simulink model "model_multicorp"  (R2026a)
settings: Solver=daessc  StopTime=0.00571428571429  MaxStep=7.93650793651e-06  RelTol=1e-9  AbsTol=1e-10
values from neighbouring files (symbols this model uses):
  C = compresor(P)    [capac.m]    (also in echilibrare.m = [0 P.r]; m02_multicorp.m = textscan(fid, ['; racire.m; s13_cinematica_fusion.m = textscan(fid, ')
  m = 3    [isg_geometrie.m]    (also in presiune_cilindru.m = u > 0 & u < 1.5)
  N = 4000    [echilibrare.m]    (also in m01_model_arbore.m = numel(th); s05_volant_activ.m = numel(th); simuleaza_arbore.m = numel(Tg))
  s = t >= t(end) - 3*60/n    [m01_model_arbore.m]    (also in racire.m = @(u) mod(-u, 360))
undefined symbols (not defined in the file or in its folder): X, Y, Z
libraries: sm_lib x21, nesl_utility x6, simulink x1
settings Model: Creator=Darian  LastModifiedBy=Darian
settings DataIOCC: OutputOption=SpecifiedOutputTimes  OutputTimes=[0 3.1746031746e-05 6.34920634921e-05 9.52380952381e-05 0.000126984126984 0.00015873015873 0.000190476190476 0.000222222222222 0.000253968253968 0.000285714285714 0.00031746031746 0.000349206349206 0.000380952380952 0.000412698412698 0.000444444444444 0.00047619047619 0.000507936507937 0.000539682539683 0.000571428571429 0.000603174603175 0.000634920634921 0.000666666666667 0.000698412698413 0.000730158730159 0.000761904761905 0.000793650793651 0.000825396825397 0.000857142857143 0.000888888888889 0.000920634920635 0.000952380952381 0.000984126984127 0.00101587301587 0.00104761904762 0.00107936507937 0.00111111111111 0.00114285714286 0.0011746031746 0.00120634920635 0.0012380952381 0.00126984126984 0.00130158730159 0.00133333333333 0.00136507936508 0.00139682539683 0.00142857142857 0.00146031746032 0.00149206349206 0.00152380952381 0.00155555555556 0.0015873015873 0.00161904761905 0.00165079365079 0.00168253968254 0.00171428571429 0.00174603174603 0.00177777777778 0.00180952380952 0.00184126984127 0.00187301587302 0.00190476190476 0.00193650793651 0.00196825396825 0.002 0.00203174603175 0.00206349206349 0.00209523809524 0.00212698412698 0.00215873015873 0.00219047619048 0.00222222222222 0.00225396825397 0.00228571428571 0.00231746031746 0.00234920634921 0.00238095238095 0.0024126984127 0.00244444444444 0.00247619047619 0.00250793650794 0.00253968253968 0.00257142857143 0.00260317460317 0.00263492063492 0.00266666666667 0.00269841269841 0.00273015873016 0.0027619047619 0.00279365079365 0.0028253968254 0.00285714285714 0.00288888888889 0.00292063492063 0.00295238095238 0.00298412698413 0.00301587301587 0.00304761904762 0.00307936507937 0.00311111111111 0.00314285714286 0.0031746031746 0.00320634920635 0.0032380952381 0.00326984126984 0.00330158730159 0.00333333333333 0.00336507936508 0.00339682539683 0.00342857142857 0.00346031746032 0.00349206349206 0.00352380952381 0.00355555555556 0.0035873015873 0.00361904761905 0.00365079365079 0.00368253968254 0.00371428571429 0.00374603174603 0.00377777777778 0.00380952380952 0.00384126984127 0.00387301587302 0.00390476190476 0.00393650793651 0.00396825396825 0.004 0.00403174603175 0.00406349206349 0.00409523809524 0.00412698412698 0.00415873015873 0.00419047619048 0.00422222222222 0.00425396825397 0.00428571428571 0.00431746031746 0.00434920634921 0.00438095238095 0.0044126984127 0.00444444444444 0.00447619047619 0.00450793650794 0.00453968253968 0.00457142857143 0.00460317460317 0.00463492063492 0.00466666666667 0.00469841269841 0.00473015873016 0.0047619047619 0.00479365079365 0.0048253968254 0.00485714285714 0.00488888888889 0.00492063492063 0.00495238095238 0.00498412698413 0.00501587301587 0.00504761904762 0.00507936507937 0.00511111111111 0.00514285714286 0.0051746031746 0.00520634920635 0.0052380952381 0.00526984126984 0.00530158730159 0.00533333333333 0.00536507936508 0.00539682539683 0.00542857142857 0.00546031746032 0.00549206349206 0.00552380952381 0.00555555555556 0.0055873015873 0.00561904761905 0.00565079365079 0.00568253968254 0.00571428571429]

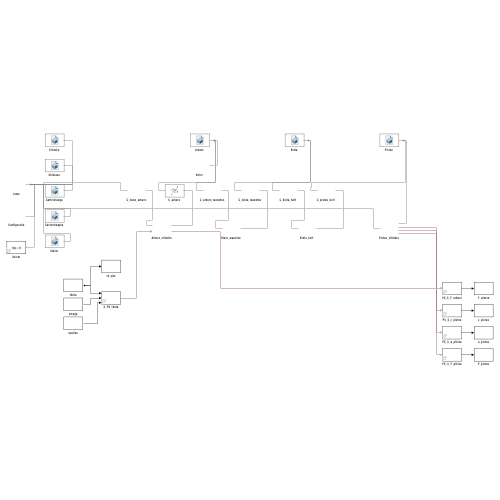
[thumbnail: Simulink's stored preview of the top-level diagram]
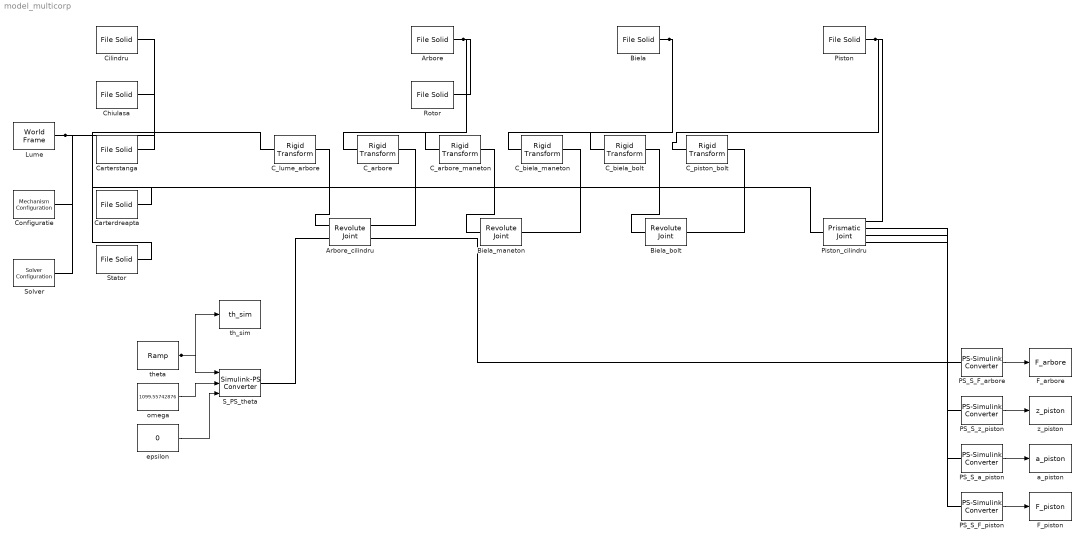
== system model_multicorp ==
  Arbore : sm_lib/Body Elements/File Solid  ExtGeomFileName=C:\Users\Darian\Documents\dizertatie_matlab\fusion\multicorp\40_Arbore.step  UnitType=FromFile  ExtGeomFileUnits=m  StepReaderType=HEX  ExportConvexHullGeometry=off  InertiaType=Custom  BasedOnType=DensityFromFile  Density=1000  DensityUnits=kg/m^3  Mass=2.277950989  MassUnits=kg  CenterOfMass=[9.035842862e-13 0.001194123027 -0.003022731061]  CenterOfMassUnits=m  MomentsOfInertia=[0.003142336917 0.001492151418 0.002716104824]  MomentsOfInertiaUnits=kg*m^2  ProductsOfInertia=[-8.580482614e-06 -8.181849604e-15 -4.711787416e-15]  ProductsOfInertiaUnits=kg*m^2  GraphicType=FromGeometry  MarkerShape=Sphere  MarkerSize=10  GraphicVisPropType=SimpleVisualProperties  GraphicDiffuseColor=[0.5 0.5 0.5]  GraphicOpacity=1  GraphicSpecularColor=[0.5 0.5 0.5 1.0]  GraphicAmbientColor=[0.15 0.15 0.15 1.0]  GraphicEmissiveColor=[0.0 0.0 0.0 1.0]  GraphicShininess=75  DoExposeReferenceFrame=on  SerializedFrames=<Frames/>
  Arbore_cilindru : sm_lib/Joints/Revolute Joint  JointMode=Normal  CompositeWrenchDir=BaseOnFollower  CompositeWrenchFrame=BaseFrame  SenseConstraintForce=off  SenseConstraintTorque=off  SenseTotalForce=on  SenseTotalTorque=off  PositionTargetSpecify=off  PositionTargetPriority=High  PositionTargetValue=0  PositionTargetValueUnits=deg  VelocityTargetSpecify=off  VelocityTargetPriority=High  VelocityTargetValue=0  VelocityTargetValueUnits=deg/s  EquilibriumPosition=0  EquilibriumPositionUnits=deg  SpringStiffness=0  SpringStiffnessUnits=N*m/deg  DampingCoefficient=0  DampingCoefficientUnits=N*m/(deg/s)  LowerLimitSpecify=off  LowerLimitBound=-90  LowerLimitBoundUnits=deg  LowerLimitStiffness=1e4  LowerLimitStiffnessUnits=N*m/deg  LowerLimitDamping=10  LowerLimitDampingUnits=N*m/(deg/s)  LowerLimitTransitionRegionWidth=0.1  LowerLimitTransitionRegionWidthUnits=deg  UpperLimitSpecify=off  UpperLimitBound=90  UpperLimitBoundUnits=deg  UpperLimitStiffness=1e4  UpperLimitStiffnessUnits=N*m/deg  UpperLimitDamping=10  UpperLimitDampingUnits=N*m/(deg/s)  UpperLimitTransitionRegionWidth=0.1  UpperLimitTransitionRegionWidthUnits=deg  TorqueActuationMode=ComputedTorque  MotionActuationMode=InputMotion  SensePosition=off  SenseVelocity=off  SenseAcceleration=off  SenseTorqueForce=off  SenseLowerLimitTorqueForce=off  SenseUpperLimitTorqueForce=off
  Biela : sm_lib/Body Elements/File Solid  ExtGeomFileName=C:\Users\Darian\Documents\dizertatie_matlab\fusion\multicorp\30_Biela.step  UnitType=FromFile  ExtGeomFileUnits=m  StepReaderType=HEX  ExportConvexHullGeometry=off  InertiaType=Custom  BasedOnType=DensityFromFile  Density=1000  DensityUnits=kg/m^3  Mass=0.181830075  MassUnits=kg  CenterOfMass=[-3.952804341e-13 -7.668919001e-19 0.0693849363]  CenterOfMassUnits=m  MomentsOfInertia=[0.0003677202797 0.0003764850798 1.5782604e-05]  MomentsOfInertiaUnits=kg*m^2  ProductsOfInertia=[-1.839056463e-20 -1.125578697e-15 -4.183320357e-21]  ProductsOfInertiaUnits=kg*m^2  GraphicType=FromGeometry  MarkerShape=Sphere  MarkerSize=10  GraphicVisPropType=SimpleVisualProperties  GraphicDiffuseColor=[0.5 0.5 0.5]  GraphicOpacity=1  GraphicSpecularColor=[0.5 0.5 0.5 1.0]  GraphicAmbientColor=[0.15 0.15 0.15 1.0]  GraphicEmissiveColor=[0.0 0.0 0.0 1.0]  GraphicShininess=75  DoExposeReferenceFrame=on  SerializedFrames=<Frames/>
  Biela_bolt : sm_lib/Joints/Revolute Joint  JointMode=Normal  CompositeWrenchDir=FollowerOnBase  CompositeWrenchFrame=BaseFrame  SenseConstraintForce=off  SenseConstraintTorque=off  SenseTotalForce=off  SenseTotalTorque=off  PositionTargetSpecify=off  PositionTargetPriority=High  PositionTargetValue=0  PositionTargetValueUnits=deg  VelocityTargetSpecify=off  VelocityTargetPriority=High  VelocityTargetValue=0  VelocityTargetValueUnits=deg/s  EquilibriumPosition=0  EquilibriumPositionUnits=deg  SpringStiffness=0  SpringStiffnessUnits=N*m/deg  DampingCoefficient=0  DampingCoefficientUnits=N*m/(deg/s)  LowerLimitSpecify=off  LowerLimitBound=-90  LowerLimitBoundUnits=deg  LowerLimitStiffness=1e4  LowerLimitStiffnessUnits=N*m/deg  LowerLimitDamping=10  LowerLimitDampingUnits=N*m/(deg/s)  LowerLimitTransitionRegionWidth=0.1  LowerLimitTransitionRegionWidthUnits=deg  UpperLimitSpecify=off  UpperLimitBound=90  UpperLimitBoundUnits=deg  UpperLimitStiffness=1e4  UpperLimitStiffnessUnits=N*m/deg  UpperLimitDamping=10  UpperLimitDampingUnits=N*m/(deg/s)  UpperLimitTransitionRegionWidth=0.1  UpperLimitTransitionRegionWidthUnits=deg  TorqueActuationMode=NoTorque  MotionActuationMode=ComputedMotion  SensePosition=off  SenseVelocity=off  SenseAcceleration=off  SenseTorqueForce=off  SenseLowerLimitTorqueForce=off  SenseUpperLimitTorqueForce=off
  Biela_maneton : sm_lib/Joints/Revolute Joint  JointMode=Normal  CompositeWrenchDir=FollowerOnBase  CompositeWrenchFrame=BaseFrame  SenseConstraintForce=off  SenseConstraintTorque=off  SenseTotalForce=off  SenseTotalTorque=off  PositionTargetSpecify=off  PositionTargetPriority=High  PositionTargetValue=0  PositionTargetValueUnits=deg  VelocityTargetSpecify=off  VelocityTargetPriority=High  VelocityTargetValue=0  VelocityTargetValueUnits=deg/s  EquilibriumPosition=0  EquilibriumPositionUnits=deg  SpringStiffness=0  SpringStiffnessUnits=N*m/deg  DampingCoefficient=0  DampingCoefficientUnits=N*m/(deg/s)  LowerLimitSpecify=off  LowerLimitBound=-90  LowerLimitBoundUnits=deg  LowerLimitStiffness=1e4  LowerLimitStiffnessUnits=N*m/deg  LowerLimitDamping=10  LowerLimitDampingUnits=N*m/(deg/s)  LowerLimitTransitionRegionWidth=0.1  LowerLimitTransitionRegionWidthUnits=deg  UpperLimitSpecify=off  UpperLimitBound=90  UpperLimitBoundUnits=deg  UpperLimitStiffness=1e4  UpperLimitStiffnessUnits=N*m/deg  UpperLimitDamping=10  UpperLimitDampingUnits=N*m/(deg/s)  UpperLimitTransitionRegionWidth=0.1  UpperLimitTransitionRegionWidthUnits=deg  TorqueActuationMode=NoTorque  MotionActuationMode=ComputedMotion  SensePosition=off  SenseVelocity=off  SenseAcceleration=off  SenseTorqueForce=off  SenseLowerLimitTorqueForce=off  SenseUpperLimitTorqueForce=off
  C_arbore : sm_lib/Frames and Transforms/Rigid Transform  RotationMethod=StandardAxis  FollAlignAxisA=+X  BaseAlignAxisA=+Y  FollAlignAxisB=+Y  BaseAlignAxisB=+Z  RotationStandardAxis=+X  RotationAngle=-90  RotationAngleUnits=deg  RotationArbitraryAxis=[0 0 1]  RotationSequenceAxes=FollowerAxes  RotationSequence=XYX  RotationSequenceAngles=[0 0 0]  RotationSequenceAnglesUnits=deg  RotationMatrix=[1 0 0;0 1 0;0 0 1]  Quaternion=[1 0 0 0]  TranslationMethod=Cartesian  TranslationCartesianOffset=[0 0 0]  TranslationCartesianOffsetUnits=m  TranslationStandardAxis=+Z  TranslationStandardOffset=0  TranslationStandardOffsetUnits=m  TranslationROffset=0  TranslationROffsetUnits=m  TranslationThetaOffset=0  TranslationThetaOffsetUnits=deg  TranslationZOffset=0  TranslationZOffsetUnits=m
  C_arbore_maneton : sm_lib/Frames and Transforms/Rigid Transform  RotationMethod=StandardAxis  FollAlignAxisA=+X  BaseAlignAxisA=+Y  FollAlignAxisB=+Y  BaseAlignAxisB=+Z  RotationStandardAxis=+X  RotationAngle=-90  RotationAngleUnits=deg  RotationArbitraryAxis=[0 0 1]  RotationSequenceAxes=FollowerAxes  RotationSequence=XYX  RotationSequenceAngles=[0 0 0]  RotationSequenceAnglesUnits=deg  RotationMatrix=[1 0 0;0 1 0;0 0 1]  Quaternion=[1 0 0 0]  TranslationMethod=Cartesian  TranslationCartesianOffset=[0 0 0.02725]  TranslationCartesianOffsetUnits=m  TranslationStandardAxis=+Z  TranslationStandardOffset=0  TranslationStandardOffsetUnits=m  TranslationROffset=0  TranslationROffsetUnits=m  TranslationThetaOffset=0  TranslationThetaOffsetUnits=deg  TranslationZOffset=0  TranslationZOffsetUnits=m
  C_biela_bolt : sm_lib/Frames and Transforms/Rigid Transform  RotationMethod=StandardAxis  FollAlignAxisA=+X  BaseAlignAxisA=+Y  FollAlignAxisB=+Y  BaseAlignAxisB=+Z  RotationStandardAxis=+X  RotationAngle=-90  RotationAngleUnits=deg  RotationArbitraryAxis=[0 0 1]  RotationSequenceAxes=FollowerAxes  RotationSequence=XYX  RotationSequenceAngles=[0 0 0]  RotationSequenceAnglesUnits=deg  RotationMatrix=[1 0 0;0 1 0;0 0 1]  Quaternion=[1 0 0 0]  TranslationMethod=Cartesian  TranslationCartesianOffset=[0 0 0.13725]  TranslationCartesianOffsetUnits=m  TranslationStandardAxis=+Z  TranslationStandardOffset=0  TranslationStandardOffsetUnits=m  TranslationROffset=0  TranslationROffsetUnits=m  TranslationThetaOffset=0  TranslationThetaOffsetUnits=deg  TranslationZOffset=0  TranslationZOffsetUnits=m
  C_biela_maneton : sm_lib/Frames and Transforms/Rigid Transform  RotationMethod=StandardAxis  FollAlignAxisA=+X  BaseAlignAxisA=+Y  FollAlignAxisB=+Y  BaseAlignAxisB=+Z  RotationStandardAxis=+X  RotationAngle=-90  RotationAngleUnits=deg  RotationArbitraryAxis=[0 0 1]  RotationSequenceAxes=FollowerAxes  RotationSequence=XYX  RotationSequenceAngles=[0 0 0]  RotationSequenceAnglesUnits=deg  RotationMatrix=[1 0 0;0 1 0;0 0 1]  Quaternion=[1 0 0 0]  TranslationMethod=Cartesian  TranslationCartesianOffset=[0 0 0.02725]  TranslationCartesianOffsetUnits=m  TranslationStandardAxis=+Z  TranslationStandardOffset=0  TranslationStandardOffsetUnits=m  TranslationROffset=0  TranslationROffsetUnits=m  TranslationThetaOffset=0  TranslationThetaOffsetUnits=deg  TranslationZOffset=0  TranslationZOffsetUnits=m
  C_lume_arbore : sm_lib/Frames and Transforms/Rigid Transform  RotationMethod=StandardAxis  FollAlignAxisA=+X  BaseAlignAxisA=+Y  FollAlignAxisB=+Y  BaseAlignAxisB=+Z  RotationStandardAxis=+X  RotationAngle=-90  RotationAngleUnits=deg  RotationArbitraryAxis=[0 0 1]  RotationSequenceAxes=FollowerAxes  RotationSequence=XYX  RotationSequenceAngles=[0 0 0]  RotationSequenceAnglesUnits=deg  RotationMatrix=[1 0 0;0 1 0;0 0 1]  Quaternion=[1 0 0 0]  TranslationMethod=Cartesian  TranslationCartesianOffset=[0 0 0]  TranslationCartesianOffsetUnits=m  TranslationStandardAxis=+Z  TranslationStandardOffset=0  TranslationStandardOffsetUnits=m  TranslationROffset=0  TranslationROffsetUnits=m  TranslationThetaOffset=0  TranslationThetaOffsetUnits=deg  TranslationZOffset=0  TranslationZOffsetUnits=m
  C_piston_bolt : sm_lib/Frames and Transforms/Rigid Transform  RotationMethod=StandardAxis  FollAlignAxisA=+X  BaseAlignAxisA=+Y  FollAlignAxisB=+Y  BaseAlignAxisB=+Z  RotationStandardAxis=+X  RotationAngle=-90  RotationAngleUnits=deg  RotationArbitraryAxis=[0 0 1]  RotationSequenceAxes=FollowerAxes  RotationSequence=XYX  RotationSequenceAngles=[0 0 0]  RotationSequenceAnglesUnits=deg  RotationMatrix=[1 0 0;0 1 0;0 0 1]  Quaternion=[1 0 0 0]  TranslationMethod=Cartesian  TranslationCartesianOffset=[0 0 0.13725]  TranslationCartesianOffsetUnits=m  TranslationStandardAxis=+Z  TranslationStandardOffset=0  TranslationStandardOffsetUnits=m  TranslationROffset=0  TranslationROffsetUnits=m  TranslationThetaOffset=0  TranslationThetaOffsetUnits=deg  TranslationZOffset=0  TranslationZOffsetUnits=m
  Carterdreapta : sm_lib/Body Elements/File Solid  ExtGeomFileName=C:\Users\Darian\Documents\dizertatie_matlab\fusion\multicorp\51_Carter_dreapta.step  UnitType=FromFile  ExtGeomFileUnits=m  StepReaderType=HEX  ExportConvexHullGeometry=off  InertiaType=Custom  BasedOnType=DensityFromFile  Density=1000  DensityUnits=kg/m^3  Mass=1  MassUnits=kg  CenterOfMass=[0 0 0]  CenterOfMassUnits=m  MomentsOfInertia=[1 1 1]*1e-3  MomentsOfInertiaUnits=kg*m^2  ProductsOfInertia=[0 0 0]  ProductsOfInertiaUnits=kg*m^2  GraphicType=FromGeometry  MarkerShape=Sphere  MarkerSize=10  GraphicVisPropType=AdvancedVisualProperties  GraphicDiffuseColor=[0.5 0.5 0.5]  GraphicOpacity=0.25  GraphicSpecularColor=[0.5 0.5 0.5 1.0]  GraphicAmbientColor=[0.15 0.15 0.15 1.0]  GraphicEmissiveColor=[0.0 0.0 0.0 1.0]  GraphicShininess=75  DoExposeReferenceFrame=on  SerializedFrames=<Frames/>
  Carterstanga : sm_lib/Body Elements/File Solid  ExtGeomFileName=C:\Users\Darian\Documents\dizertatie_matlab\fusion\multicorp\50_Carter_stanga.step  UnitType=FromFile  ExtGeomFileUnits=m  StepReaderType=HEX  ExportConvexHullGeometry=off  InertiaType=Custom  BasedOnType=DensityFromFile  Density=1000  DensityUnits=kg/m^3  Mass=1  MassUnits=kg  CenterOfMass=[0 0 0]  CenterOfMassUnits=m  MomentsOfInertia=[1 1 1]*1e-3  MomentsOfInertiaUnits=kg*m^2  ProductsOfInertia=[0 0 0]  ProductsOfInertiaUnits=kg*m^2  GraphicType=FromGeometry  MarkerShape=Sphere  MarkerSize=10  GraphicVisPropType=AdvancedVisualProperties  GraphicDiffuseColor=[0.5 0.5 0.5]  GraphicOpacity=0.25  GraphicSpecularColor=[0.5 0.5 0.5 1.0]  GraphicAmbientColor=[0.15 0.15 0.15 1.0]  GraphicEmissiveColor=[0.0 0.0 0.0 1.0]  GraphicShininess=75  DoExposeReferenceFrame=on  SerializedFrames=<Frames/>
  Chiulasa : sm_lib/Body Elements/File Solid  ExtGeomFileName=C:\Users\Darian\Documents\dizertatie_matlab\fusion\multicorp\15_Chiulasa.step  UnitType=FromFile  ExtGeomFileUnits=m  StepReaderType=HEX  ExportConvexHullGeometry=off  InertiaType=Custom  BasedOnType=DensityFromFile  Density=1000  DensityUnits=kg/m^3  Mass=1  MassUnits=kg  CenterOfMass=[0 0 0]  CenterOfMassUnits=m  MomentsOfInertia=[1 1 1]*1e-3  MomentsOfInertiaUnits=kg*m^2  ProductsOfInertia=[0 0 0]  ProductsOfInertiaUnits=kg*m^2  GraphicType=FromGeometry  MarkerShape=Sphere  MarkerSize=10  GraphicVisPropType=AdvancedVisualProperties  GraphicDiffuseColor=[0.5 0.5 0.5]  GraphicOpacity=0.25  GraphicSpecularColor=[0.5 0.5 0.5 1.0]  GraphicAmbientColor=[0.15 0.15 0.15 1.0]  GraphicEmissiveColor=[0.0 0.0 0.0 1.0]  GraphicShininess=75  DoExposeReferenceFrame=on  SerializedFrames=<Frames/>
  Cilindru : sm_lib/Body Elements/File Solid  ExtGeomFileName=C:\Users\Darian\Documents\dizertatie_matlab\fusion\multicorp\10_Cilindru.step  UnitType=FromFile  ExtGeomFileUnits=m  StepReaderType=HEX  ExportConvexHullGeometry=off  InertiaType=Custom  BasedOnType=DensityFromFile  Density=1000  DensityUnits=kg/m^3  Mass=1  MassUnits=kg  CenterOfMass=[0 0 0]  CenterOfMassUnits=m  MomentsOfInertia=[1 1 1]*1e-3  MomentsOfInertiaUnits=kg*m^2  ProductsOfInertia=[0 0 0]  ProductsOfInertiaUnits=kg*m^2  GraphicType=FromGeometry  MarkerShape=Sphere  MarkerSize=10  GraphicVisPropType=AdvancedVisualProperties  GraphicDiffuseColor=[0.5 0.5 0.5]  GraphicOpacity=0.25  GraphicSpecularColor=[0.5 0.5 0.5 1.0]  GraphicAmbientColor=[0.15 0.15 0.15 1.0]  GraphicEmissiveColor=[0.0 0.0 0.0 1.0]  GraphicShininess=75  DoExposeReferenceFrame=on  SerializedFrames=<Frames/>
  Configuratie : sm_lib/Utilities/Mechanism Configuration  UniformGravity=None  GravityVector=[0 0 -9.80665]  GravityVectorUnits=m/s^2  LinearizationDelta=0.001  JointModeTransitionNonlinearIterations=2
  F_arbore : ToWorkspace  VariableName=F_arbore  SampleTime=-1
  F_piston : ToWorkspace  VariableName=F_piston  SampleTime=-1
  Lume : sm_lib/Frames and Transforms/World Frame
  PS_S_F_arbore : nesl_utility/PS-Simulink Converter  PhysicalDomain=network_engine_domain  SubClassName=ps_output  LeftPortType=input  RightPortType=output  PseudoPeriodic=off  Frequencies=[]  VectorFormat=inherit  Unit=N  AffineConversion=off
  PS_S_F_piston : nesl_utility/PS-Simulink Converter  PhysicalDomain=network_engine_domain  SubClassName=ps_output  LeftPortType=input  RightPortType=output  PseudoPeriodic=off  Frequencies=[]  VectorFormat=inherit  Unit=N  AffineConversion=off
  PS_S_a_piston : nesl_utility/PS-Simulink Converter  PhysicalDomain=network_engine_domain  SubClassName=ps_output  LeftPortType=input  RightPortType=output  PseudoPeriodic=off  Frequencies=[]  VectorFormat=inherit  Unit=m/s^2  AffineConversion=off
  PS_S_z_piston : nesl_utility/PS-Simulink Converter  PhysicalDomain=network_engine_domain  SubClassName=ps_output  LeftPortType=input  RightPortType=output  PseudoPeriodic=off  Frequencies=[]  VectorFormat=inherit  Unit=m  AffineConversion=off
  Piston : sm_lib/Body Elements/File Solid  ExtGeomFileName=C:\Users\Darian\Documents\dizertatie_matlab\fusion\multicorp\20_Piston.step  UnitType=FromFile  ExtGeomFileUnits=m  StepReaderType=HEX  ExportConvexHullGeometry=off  InertiaType=Custom  BasedOnType=DensityFromFile  Density=1000  DensityUnits=kg/m^3  Mass=0.185436751097  MassUnits=kg  CenterOfMass=[6.905124872e-12 -1.21802503e-17 0.1414924909]  CenterOfMassUnits=m  MomentsOfInertia=[8.483689436e-05 7.17072313e-05 7.200721919e-05]  MomentsOfInertiaUnits=kg*m^2  ProductsOfInertia=[9.179246487e-21 1.443561615e-14 -7.617018129e-20]  ProductsOfInertiaUnits=kg*m^2  GraphicType=FromGeometry  MarkerShape=Sphere  MarkerSize=10  GraphicVisPropType=SimpleVisualProperties  GraphicDiffuseColor=[0.5 0.5 0.5]  GraphicOpacity=1  GraphicSpecularColor=[0.5 0.5 0.5 1.0]  GraphicAmbientColor=[0.15 0.15 0.15 1.0]  GraphicEmissiveColor=[0.0 0.0 0.0 1.0]  GraphicShininess=75  DoExposeReferenceFrame=on  SerializedFrames=<Frames/>
  Piston_cilindru : sm_lib/Joints/Prismatic Joint  JointMode=Normal  CompositeWrenchDir=BaseOnFollower  CompositeWrenchFrame=BaseFrame  SenseConstraintForce=off  SenseConstraintTorque=off  SenseTotalForce=on  SenseTotalTorque=off  PositionTargetSpecify=off  PositionTargetPriority=High  PositionTargetValue=0  PositionTargetValueUnits=m  VelocityTargetSpecify=off  VelocityTargetPriority=High  VelocityTargetValue=0  VelocityTargetValueUnits=m/s  EquilibriumPosition=0  EquilibriumPositionUnits=m  SpringStiffness=0  SpringStiffnessUnits=N/m  DampingCoefficient=0  DampingCoefficientUnits=N/(m/s)  LowerLimitSpecify=off  LowerLimitBound=-1  LowerLimitBoundUnits=m  LowerLimitStiffness=1e6  LowerLimitStiffnessUnits=N/m  LowerLimitDamping=1e3  LowerLimitDampingUnits=N/(m/s)  LowerLimitTransitionRegionWidth=1e-4  LowerLimitTransitionRegionWidthUnits=m  UpperLimitSpecify=off  UpperLimitBound=1  UpperLimitBoundUnits=m  UpperLimitStiffness=1e6  UpperLimitStiffnessUnits=N/m  UpperLimitDamping=1e3  UpperLimitDampingUnits=N/(m/s)  UpperLimitTransitionRegionWidth=1e-4  UpperLimitTransitionRegionWidthUnits=m  TorqueActuationMode=NoTorque  MotionActuationMode=ComputedMotion  SensePosition=on  SenseVelocity=off  SenseAcceleration=on  SenseTorqueForce=off  SenseLowerLimitTorqueForce=off  SenseUpperLimitTorqueForce=off
  Rotor : sm_lib/Body Elements/File Solid  ExtGeomFileName=C:\Users\Darian\Documents\dizertatie_matlab\fusion\multicorp\61_Rotor.step  UnitType=FromFile  ExtGeomFileUnits=m  StepReaderType=HEX  ExportConvexHullGeometry=off  InertiaType=Custom  BasedOnType=DensityFromFile  Density=1000  DensityUnits=kg/m^3  Mass=1.295359192  MassUnits=kg  CenterOfMass=[-4.302855319e-15 -0.06803257502 -2.037018277e-06]  CenterOfMassUnits=m  MomentsOfInertia=[0.002051694145 0.003836204031 0.002051738113]  MomentsOfInertiaUnits=kg*m^2  ProductsOfInertia=[-4.709618077e-09 3.10939897e-18 -7.902195499e-17]  ProductsOfInertiaUnits=kg*m^2  GraphicType=FromGeometry  MarkerShape=Sphere  MarkerSize=10  GraphicVisPropType=SimpleVisualProperties  GraphicDiffuseColor=[0.5 0.5 0.5]  GraphicOpacity=1  GraphicSpecularColor=[0.5 0.5 0.5 1.0]  GraphicAmbientColor=[0.15 0.15 0.15 1.0]  GraphicEmissiveColor=[0.0 0.0 0.0 1.0]  GraphicShininess=75  DoExposeReferenceFrame=on  SerializedFrames=<Frames/>
  S_PS_theta : nesl_utility/Simulink-PS Converter  PhysicalDomain=network_engine_domain  SubClassName=ps_input  LeftPortType=input  RightPortType=output  PseudoPeriodic=off  Frequencies=[]  NoiseDistribution=none  NoiseParameters=[]  Unit=rad  AffineConversion=off  FilteringAndDerivatives=provide  SimscapeFilterOrder=1  InputFilterTimeConstant=0.001  UdotUserProvided=2
  Solver : nesl_utility/Solver Configuration  PhysicalDomain=network_engine_domain  SubClassName=solver  LeftPortType=input  RightPortType=generic  Tones=[]  Harmonics=[]  SimulateNoise=off  Profile=off  UseLocalSampling=off  EnableSwitchedLinearOptims=on  FrequencyDomain=off  UseCCode=off  RelTol=0.001  AbsTol=0.001  MinStep=1e-09  ToWorkspace=off  RevertToSquareIcSolve=off  NumHomotopyIterations=100  PhasorMode=off  PhasorModeNumHarmonics=1  ConsistencySolver=NEWTON_XTOL_AFTER_FTOL  CanonicalOrdering=CANONICAL  OptimizeIntermediates=OPTIMIZED  IndexReductionMethod=DerivativeReplacement  DoDC=off  ResidualTolerance=1e-09  ConsistencyTolSource=GLOBAL  ConsistencyAbsTol=0.001  ConsistencyRelTol=0.001  ConsistencyTolFactor=0.001  UseLocalSolver=off  LocalSolverChoice=NE_BACKWARD_EULER_ADVANCER  ResolveIndetEquations=on  FunctionEvalNumThread=1  LocalSolverSampleTime=0.001  DoFixedCost=off  MaxNonlinIter=3  MaxModeIter=2  ComputeImpulses=off  ImpulseIterations=2  LinearAlgebra=auto  LinearAlgebraNumThread=0  EquationFormulation=NE_TIME_EF  DelaysMemoryBudget=1024  AutomaticFiltering=on  FilteringTimeConstant=0.001  PartitionStorageMethod=AS_NEEDED  PartitionMemoryBudget=1024  PartitionMethod=ROBUST  MultibodyUseLocalSolver=off  MultibodyLocalSolverChoice=ODE1  MultibodyLocalSolverSampleTime=0.001
  Stator : sm_lib/Body Elements/File Solid  ExtGeomFileName=C:\Users\Darian\Documents\dizertatie_matlab\fusion\multicorp\60_Stator.step  UnitType=FromFile  ExtGeomFileUnits=m  StepReaderType=HEX  ExportConvexHullGeometry=off  InertiaType=Custom  BasedOnType=DensityFromFile  Density=1000  DensityUnits=kg/m^3  Mass=1  MassUnits=kg  CenterOfMass=[0 0 0]  CenterOfMassUnits=m  MomentsOfInertia=[1 1 1]*1e-3  MomentsOfInertiaUnits=kg*m^2  ProductsOfInertia=[0 0 0]  ProductsOfInertiaUnits=kg*m^2  GraphicType=FromGeometry  MarkerShape=Sphere  MarkerSize=10  GraphicVisPropType=AdvancedVisualProperties  GraphicDiffuseColor=[0.5 0.5 0.5]  GraphicOpacity=0.25  GraphicSpecularColor=[0.5 0.5 0.5 1.0]  GraphicAmbientColor=[0.15 0.15 0.15 1.0]  GraphicEmissiveColor=[0.0 0.0 0.0 1.0]  GraphicShininess=75  DoExposeReferenceFrame=on  SerializedFrames=<Frames/>
  a_piston : ToWorkspace  VariableName=a_piston  SampleTime=-1
  epsilon : Constant  Value=0
  omega : Constant  Value=1099.55742876
  th_sim : ToWorkspace  VariableName=th_sim  SampleTime=-1
  theta : simulink/Sources/Ramp  slope=1099.55742876  start=0  InitialOutput=0
  z_piston : ToWorkspace  VariableName=z_piston  SampleTime=-1
  wires:
  theta/1 -> S_PS_theta/1, th_sim/1
  omega/1 -> S_PS_theta/2
  epsilon/1 -> S_PS_theta/3
  PS_S_F_arbore/1 -> F_arbore/1
  PS_S_z_piston/1 -> z_piston/1
  PS_S_a_piston/1 -> a_piston/1
  PS_S_F_piston/1 -> F_piston/1
  connections:
  Configuratie/RConn1 -- Lume/RConn1 -- Solver/RConn1 -- Cilindru/RConn1 -- Chiulasa/RConn1 -- Carterstanga/RConn1 -- Carterdreapta/RConn1 -- Stator/RConn1 -- C_lume_arbore/LConn1 -- Piston_cilindru/LConn1
  Rotor/RConn1 -- C_arbore/LConn1 -- Arbore/RConn1 -- C_arbore_maneton/LConn1
  C_biela_maneton/LConn1 -- Biela/RConn1 -- C_biela_bolt/LConn1
  C_piston_bolt/LConn1 -- Piston/RConn1 -- Piston_cilindru/RConn1
  C_lume_arbore/RConn1 -- Arbore_cilindru/LConn1
  Arbore_cilindru/RConn1 -- C_arbore/RConn1
  C_arbore_maneton/RConn1 -- Biela_maneton/LConn1
  Biela_maneton/RConn1 -- C_biela_maneton/RConn1
  C_biela_bolt/RConn1 -- Biela_bolt/LConn1
  Biela_bolt/RConn1 -- C_piston_bolt/RConn1
  S_PS_theta/RConn1 -- Arbore_cilindru/LConn2
  Arbore_cilindru/RConn2 -- PS_S_F_arbore/LConn1
  Piston_cilindru/RConn2 -- PS_S_z_piston/LConn1
  Piston_cilindru/RConn3 -- PS_S_a_piston/LConn1
  Piston_cilindru/RConn4 -- PS_S_F_piston/LConn1
